simulink model "orig_exp3_feedback"  (R2023a)
settings: Solver=ode4  StartTime=0.0  StopTime=20  FixedStep=0.001  RelTol=1e-3
settings Model: Creator=Anonymous  LastModifiedBy=Anonymous

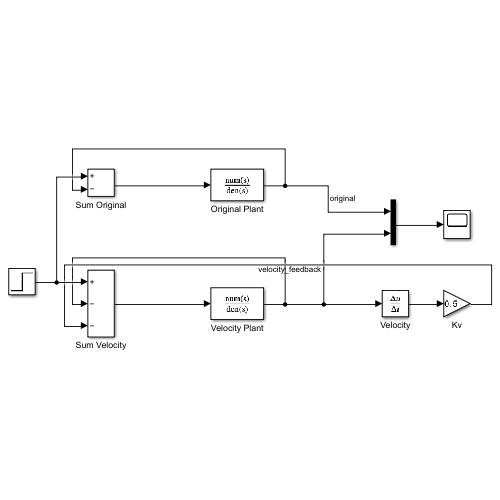
[thumbnail: Simulink's stored preview of the top-level diagram]
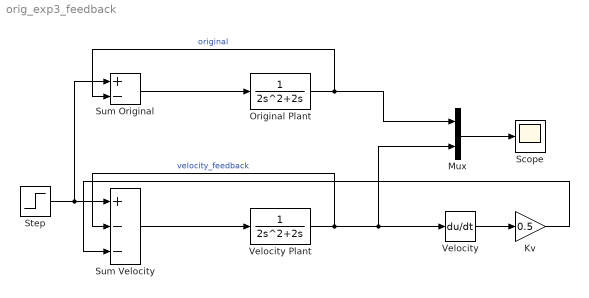
== system orig_exp3_feedback ==
  Kv : Gain  Gain=0.5
  Mux : Mux  Inputs=2
  Original Plant : TransferFcn  Numerator=1  Denominator=[2 2 0]
  Scope : Scope
  Step : Step  Time=0  SampleTime=0
  Sum Original : Sum  Inputs=+-
  Sum Velocity : Sum  Inputs=+--
  Velocity : Derivative
  Velocity Plant : TransferFcn  Numerator=1  Denominator=[2 2 0]
  wires:
  Mux/1 -> Scope/1
  Kv/1 -> Sum Velocity/3
  Velocity/1 -> Kv/1
  Velocity Plant/1 -> Mux/2, Velocity/1, Sum Velocity/2  "velocity_feedback"
  Sum Velocity/1 -> Velocity Plant/1
  Original Plant/1 -> Mux/1, Sum Original/2  "original"
  Sum Original/1 -> Original Plant/1
  Step/1 -> Sum Velocity/1, Sum Original/1
